simulink subsystem "Parking"  (R2024a)
settings: Solver=VariableStepAuto  StartTime=0.0  StopTime=10.0  RelTol=1e-3
settings Model: Creator=User  LastModifiedBy=User

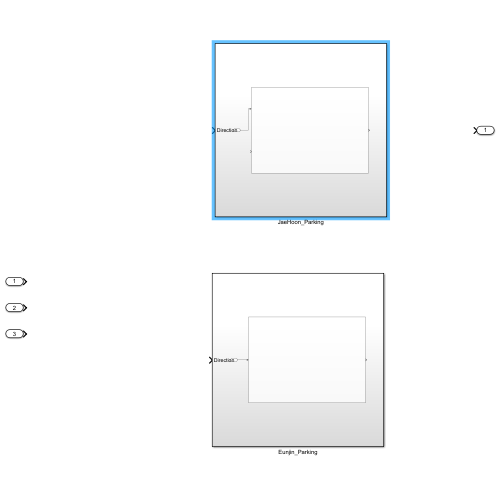
[thumbnail: Simulink's stored preview of the top-level diagram]
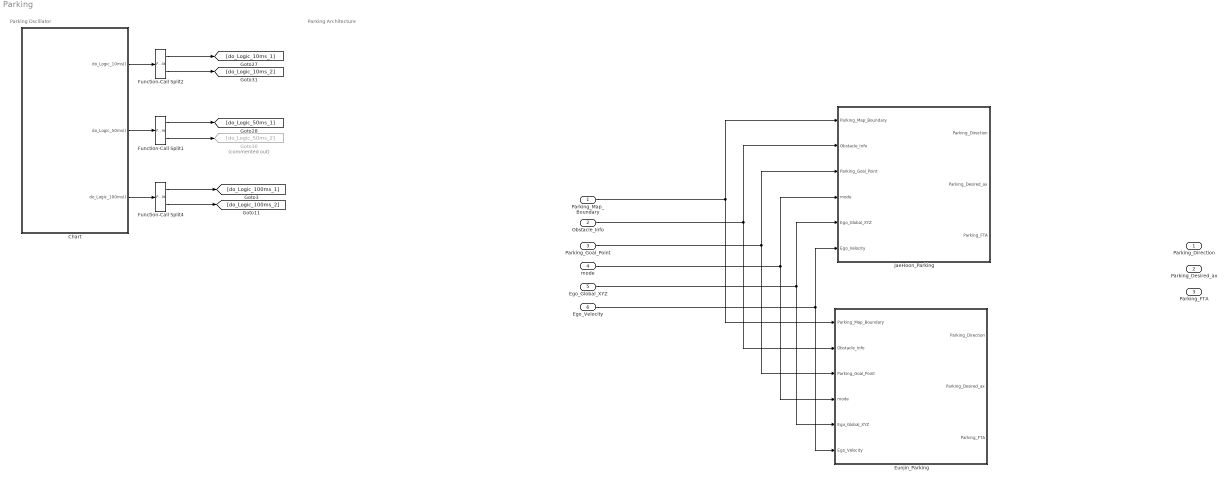
== system Parking ==
  note: Parking Oscillator
  note: Parking Architecture
  Parking_Map_Boundary : Inport
  Obstacle_Info : Inport  Port=2
  Parking_Goal_Point : Inport  Port=3
  mode : Inport  Port=4
  Ego_Global_XYZ : Inport  Port=5
  Ego_Velocity : Inport  Port=6
  Chart : Stateflow chart  TreatAsAtomicUnit=on
  Eunjin_Parking : Subsystem
  Function-Call Split1 : FunctionCallSplit  IconShape=distinctive  NumOutputPorts=2  OutputPortLayout=default
  Function-Call Split2 : FunctionCallSplit  IconShape=distinctive  NumOutputPorts=2  OutputPortLayout=default
  Function-Call Split4 : FunctionCallSplit  IconShape=distinctive  NumOutputPorts=2  OutputPortLayout=default
  Goto30 : Goto  Commented=on  GotoTag=do_Logic_50ms_2
  JaeHoon_Parking : Subsystem
  Parking_Direction : Outport
  Parking_Desired_ax : Outport  Port=2
  Parking_FTA : Outport  Port=3
  wires:
  Parking_Map_Boundary/1 -> JaeHoon_Parking/1(Parking_Map_Boundary), Eunjin_Parking/1(Parking_Map_Boundary)
  Obstacle_Info/1 -> JaeHoon_Parking/2(Obstacle_Info), Eunjin_Parking/2(Obstacle_Info)
  Parking_Goal_Point/1 -> Eunjin_Parking/3(Parking_Goal_Point), JaeHoon_Parking/3(Parking_Goal_Point)
  mode/1 -> JaeHoon_Parking/4(mode), Eunjin_Parking/4(mode)
  Ego_Global_XYZ/1 -> JaeHoon_Parking/5(Ego_Global_XYZ), Eunjin_Parking/5(Ego_Global_XYZ)
  Ego_Velocity/1 -> Eunjin_Parking/6(Ego_Velocity), JaeHoon_Parking/6(Ego_Velocity)
  Chart/1(do_Logic_10ms()) -> Function-Call Split2/1
  Function-Call Split2/1 -> [do_Logic_10ms_1]
  Function-Call Split4/1 -> [do_Logic_100ms_1]
  Function-Call Split4/2 -> [do_Logic_100ms_2]
  Chart/3(do_Logic_100ms()) -> Function-Call Split4/1
  Function-Call Split2/2 -> [do_Logic_10ms_2]
  Function-Call Split1/2 -> Goto30/1
  Function-Call Split1/1 -> [do_Logic_50ms_1]
  Chart/2(do_Logic_50ms()) -> Function-Call Split1/1

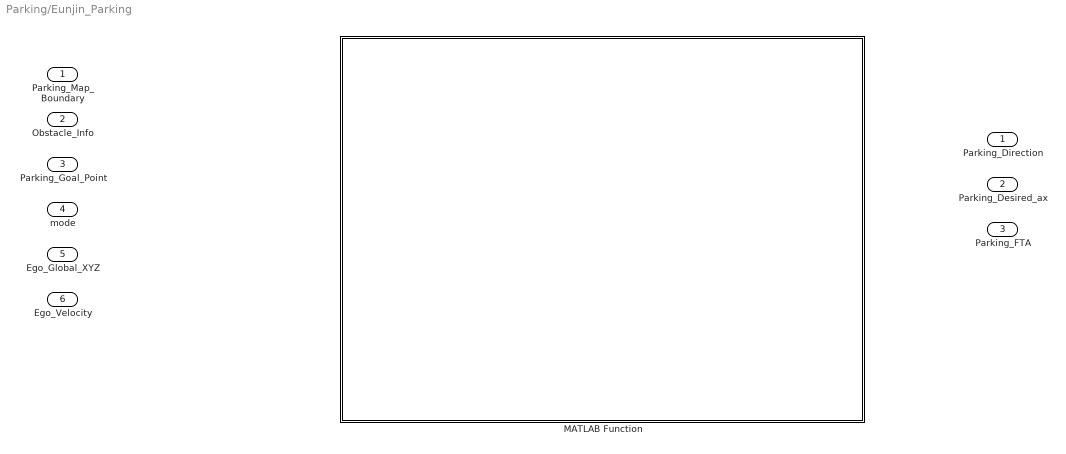
== system Parking/Eunjin_Parking ==
  Parking_Map_Boundary : Inport
  Obstacle_Info : Inport  Port=2
  Parking_Goal_Point : Inport  Port=3
  mode : Inport  Port=4
  Ego_Global_XYZ : Inport  Port=5
  Ego_Velocity : Inport  Port=6
  MATLAB Function : MATLAB Function  TreatAsAtomicUnit=on
  Parking_Direction : Outport
  Parking_Desired_ax : Outport  Port=2
  Parking_FTA : Outport  Port=3

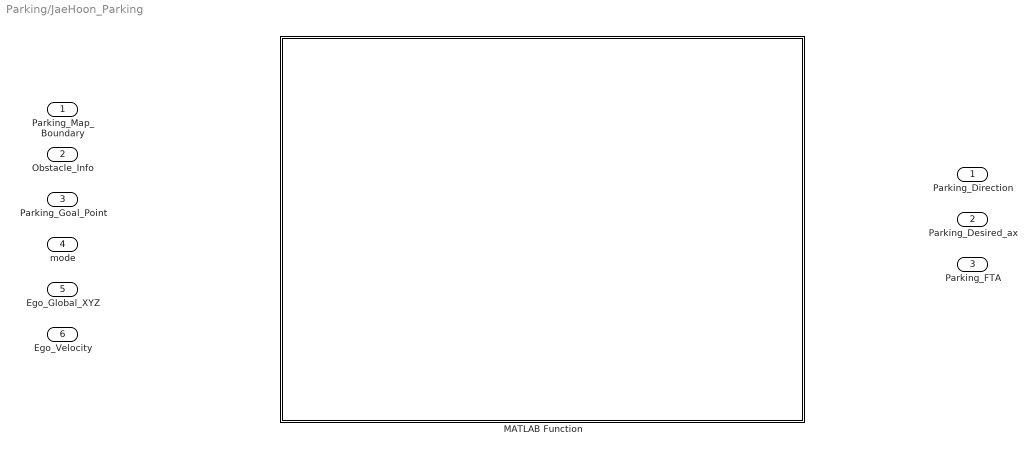
== system Parking/JaeHoon_Parking ==
  Parking_Map_Boundary : Inport
  Obstacle_Info : Inport  Port=2
  Parking_Goal_Point : Inport  Port=3
  mode : Inport  Port=4
  Ego_Global_XYZ : Inport  Port=5
  Ego_Velocity : Inport  Port=6
  MATLAB Function : MATLAB Function  TreatAsAtomicUnit=on
  Parking_Direction : Outport
  Parking_Desired_ax : Outport  Port=2
  Parking_FTA : Outport  Port=3

== matlab function Parking/Eunjin_Parking/MATLAB Function ==
function Parking
asfdasfasdfd
y = u;

== matlab function Parking/JaeHoon_Parking/MATLAB Function ==
function Parking
asfdasfasdfd
y = u;

== stateflow chart Parking/Chart ==
  (default) -> (junction 1)
  (junction 1) -> (junction 3) [order 1] : [mod(i,10) == 0]
      | {do_Logic_10ms;}
  (junction 1) -> (junction 7) [order 2]
  (junction 3) -> (junction 5)
  (junction 5) -> (junction 7)
  (junction 7) -> (junction 10)
  (junction 10) -> (junction 12) [order 1] : [mod(i, 50) == 0]
      | {do_Logic_50ms;}
  (junction 10) -> (junction 18) [order 2]
  (junction 12) -> (junction 16)
  (junction 16) -> (junction 18)
  (junction 18) -> (junction 25)
  (junction 25) -> (junction 27) [order 1] : [mod(i,100) == 0]
      | {do_Logic_100ms;}
  (junction 25) -> (junction 21) [order 2]
  (junction 27) -> (junction 29) : {i = 0;}
  (junction 29) -> (junction 21)
  (junction 21) -> (junction 32) : {i = i +1;}
  data: i local =0
  events: do_Logic_10ms output FUNCTION_CALL_EVENT; do_Logic_50ms output FUNCTION_CALL_EVENT; do_Logic_100ms output FUNCTION_CALL_EVENT
